simulink model "sens_acq_lidar"  (R2026b)
settings: Solver=VariableStepAuto
values from neighbouring files (symbols this model uses):
  P = (P + P.')/2    [sens_nav_ekf.m]
undefined symbols (not defined in the file or in its folder): sens_per_prm, Ts
settings Model: Creator=aomar  LastModifiedBy=aomar

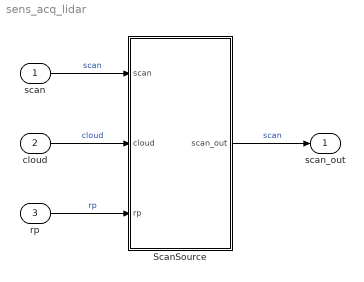
== system sens_acq_lidar ==
  scan : Inport  OutDataTypeStr=Bus: Bus_LidarScanRaw  SampleTime=Ts.lidar
  cloud : Inport  Port=2  OutDataTypeStr=Bus: Bus_LidarCloudRaw  SampleTime=Ts.lidar
  rp : Inport  Port=3  OutDataTypeStr=double  PortDimensions=2  SampleTime=Ts.lidar
  ScanSource : Subsystem  Variant=on
  scan_out : Outport  OutDataTypeStr=Bus: Bus_LidarScanRaw
  wires:
  scan/1 -> ScanSource/1(scan)  "scan"
  cloud/1 -> ScanSource/2(cloud)  "cloud"
  rp/1 -> ScanSource/3(rp)  "rp"
  ScanSource/1(scan_out) -> scan_out/1  "scan"

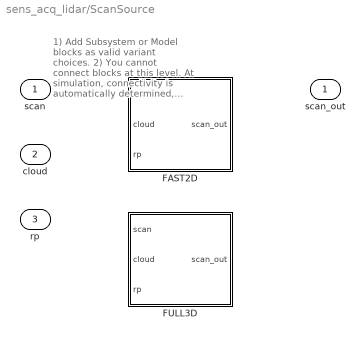
== system sens_acq_lidar/ScanSource ==
  note: 1) Add Subsystem or Model blocks as valid variant choices.
      | 2) You cannot connect blocks at this level. At simulation, connectivity is automatically
      | determined, based on the active variant and port name matching.
  scan : Inport
  cloud : Inport  Port=2
  rp : Inport  Port=3
  FAST2D : Subsystem  Description=FAST2D (VC_LIDAR == 1): the plant 360-beam scan is passed through.  VariantControl=VC_LIDAR == 1
  FULL3D : Subsystem  Description=FULL3D (VC_LIDAR == 2): organised cloud (Bus_LidarCloudRaw) -> MATLAB Function sens_lidar_cloud2scan (F4) -> Bus_LidarScanRaw.  VariantControl=VC_LIDAR == 2
  scan_out : Outport

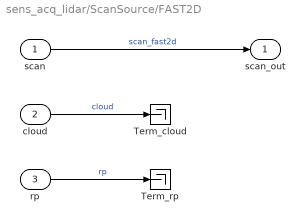
== system sens_acq_lidar/ScanSource/FAST2D ==
  scan : Inport
  cloud : Inport  Port=2
  rp : Inport  Port=3
  Term_cloud : Terminator
  Term_rp : Terminator
  scan_out : Outport
  wires:
  scan/1 -> scan_out/1  "scan_fast2d"
  cloud/1 -> Term_cloud/1  "cloud"
  rp/1 -> Term_rp/1  "rp"

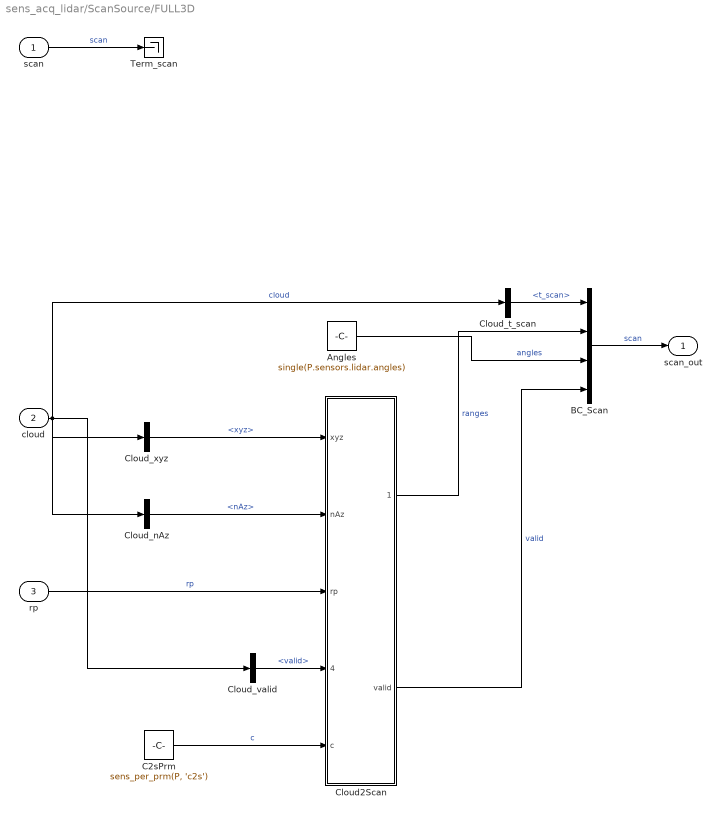
== system sens_acq_lidar/ScanSource/FULL3D ==
  scan : Inport
  cloud : Inport  Port=2
  rp : Inport  Port=3
  Angles : Constant  Value=single(P.sensors.lidar.angles)  OutDataTypeStr=single  SampleTime=Ts.lidar
  BC_Scan : BusCreator  Inputs=4  OutDataTypeStr=Bus: Bus_LidarScanRaw  NonVirtualBus=on
      settings: InheritFromInputs=off
  C2sPrm : Constant  Value=sens_per_prm(P, 'c2s')
  Cloud2Scan : MATLAB Function  TreatAsAtomicUnit=on
  Cloud_nAz : BusSelector  OutputSignals=nAz
  Cloud_t_scan : BusSelector  OutputSignals=t_scan
  Cloud_valid : BusSelector  OutputSignals=valid
  Cloud_xyz : BusSelector  OutputSignals=xyz
  Term_scan : Terminator
  scan_out : Outport
  wires:
  scan/1 -> Term_scan/1  "scan"
  cloud/1 -> Cloud_valid/1, Cloud_t_scan/1, Cloud_nAz/1, Cloud_xyz/1  "cloud"
  rp/1 -> Cloud2Scan/3(rp)  "rp"
  Cloud_xyz/1 -> Cloud2Scan/1(xyz)  "<xyz>"
  Cloud_nAz/1 -> Cloud2Scan/2(nAz)  "<nAz>"
  C2sPrm/1 -> Cloud2Scan/5(c)  "c"
  Cloud_valid/1 -> Cloud2Scan/4(cloudValid)  "<valid>"
  Angles/1 -> BC_Scan/3  "angles"
  Cloud2Scan/1(ranges) -> BC_Scan/2  "ranges"
  Cloud2Scan/2(valid) -> BC_Scan/4  "valid"
  Cloud_t_scan/1 -> BC_Scan/1  "<t_scan>"
  BC_Scan/1 -> scan_out/1  "scan"

== matlab function sens_acq_lidar/ScanSource/FULL3D/Cloud2Scan ==
  settings: description=Cloud -> 360-beam height-band scan (sensors spec 3.4 / F4): subsystems/sensors/sens_lidar_cloud2scan.m; constants on input 5 (sens_per_prm(P, 'c2s'))
  data: xyz input; ranges output; nAz input; rp input; cloudValid input; c input; valid output
function [ranges, valid] = fcn(xyz, nAz, rp, cloudValid, c)
%#codegen
[ranges, valid] = sens_lidar_cloud2scan(xyz, nAz, rp, cloudValid, c);
